simulink model "scalar_const_noise"  (Simulink 5.0)
settings: Solver=ode45  StartTime=0.0  StopTime=1000.0  RelTol=1e-3
libraries: simulink x1
settings Model: Creator=mcarroll  LastModifiedBy=mcarroll  ExtModeAutoUpdateStatusClock=off  BlockReductionOpt=off  BooleanDataType=off

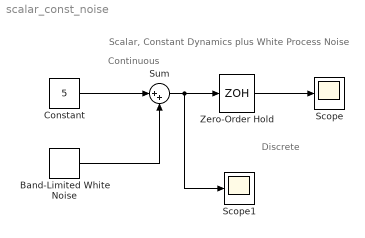
== system scalar_const_noise ==
  note: Scalar, Constant Dynamics
      | plus White Process Noise
  note: Continuous
  note: Discrete
  Band-Limited White Noise : simulink/Sources/Band-Limited White Noise  Cov=[0.1]  Ts=0.1  seed=[floor(rand*100)+23341]
  Constant : Constant  Value=5
  Scope : Scope
      settings: YMin=3  YMax=8
  Scope1 : Scope
      settings: YMin=3  YMax=8
  Sum : Sum  Inputs=|++  SaturateOnIntegerOverflow=on  InputSameDT=on
  Zero-Order Hold : ZeroOrderHold  SampleTime=2
  wires:
  Band-Limited White Noise/1 -> Sum/2
  Constant/1 -> Sum/1
  Sum/1 -> Zero-Order Hold/1, Scope1/1
  Zero-Order Hold/1 -> Scope/1
